simulink model "testrig_toe_camber_caster_kpi"  (R2024b)
settings: Solver=ode23t  StartTime=0.0  StopTime=309  MaxStep=0.01  RelTol=1e-3  AbsTol=1e-3  EnableMultiTasking=on
PostLoadFcn:
  | Maneuver = MDatabase.KnC.Sedan_HambaLG;
values from neighbouring files (symbols this model uses):
  Vehicle = evalin('base','Vehicle')    [sm_car_knc_plot1toecamber.m]    (also in testrig_quarter_car_results.m = sm_car_vehcfg_setPeopleOnOff(Vehicle,[0 0 0 0 0],'SuspA1'))
undefined symbols (not defined in the file or in its folder): X, Y, Z
libraries: sm_lib x12, sm_car_testrig_utilities_lib x5, nesl_utility x3, Suspension_Utilities x1
settings Model: Creator=smiller  LastModifiedBy=smiller
settings SolverCC: AutoScaleAbsTol=off  AlgebraicLoopSolver=TrustRegion  MaxZcPerStep=1
settings DataIOCC: LimitDataPoints=on  MaxDataPoints=10000  ReturnWorkspaceOutputs=off  SignalLoggingName=logsout_sm_car_testrig_quarter_car
settings OptimizationCC: LifeSpan=inf
settings DebuggingCC: UnconnectedInputMsg=warning  UnconnectedOutputMsg=warning  UnconnectedLineMsg=warning  AllowSymbolicDim=off  SFUnexpectedBacktrackingDiag=warning  SFNoUnconditionalDefaultTransitionDiag=warning  SFExecutionAtInitializationDiag=none  ArithmeticOperatorsInVariantConditions=warning
settings ModelReferenceCC: EnableRefExpFcnMdlSchedulingChecks=on
settings SFSimCC: SimUseLocalCustomCode=off  CustomCodeUndefinedFunction=UseInterfaceOnly
settings RTWCC: RTWUseLocalCustomCode=off  GPUComputeCapability=3.5  DLArmComputeVersion=19.05
settings CodeAppCC: StateflowObjectComments=on
settings GRTTargetCC: TargetLangStandard=C89/C90 (ANSI)
settings ConfigComp: CovMetricSettings=dw  CovSaveCumulativeToWorkspaceVar=on  CovSaveSingleToWorkspaceVar=on  CovExternalEMLEnable=off  CovSFcnEnable=off
settings SimscapeCC: SimscapeLogType=all  SimscapeLogSimulationStatistics=on  SimscapeLogName=simlog_sm_car_testrig_quarter_car  SimscapeLogLimitData=off  SimscapeLogDataHistory=10000
settings ExplorerConfigSet: InternalSimMechanicsExplorerSettings="<ExplorerConfiguration><canonicalview>default</canonicalview><AnimationSetting><BasePlaybackSpeed>1.0</BasePlaybackSpeed><PlaybackSpeedFactor>16.0</PlaybackSpeedFactor></AnimationSetting><TilePanel><TileInfo><Tiles Columns=\"2\" Count=\"4\" Rows=\"2\"><Column Weight=\"0.4994\"/><Column Weight=\"0.5006\"/><Row Weight=\"0.5\"/><Row Weight=\"0.5\"/><Tile Height=\"1\" Width=\"1\" X=\"0\" Y=\"0\"/><Tile Height=\"1\" Width=\"1\" X=\"0\" Y=\"1\"/><Tile Height=\"1\" Width=\"1\" X=\"1\" Y=\"0\"/><Tile Height=\"1\" Width=\"1\" X=\"1\" Y=\"1\"/></Tiles></TileInfo><SceneInfo><SceneViewer><BGColor><R>0.60000002384185791</R><G>0.60000002384185791</G><B>0.60000002384185791</B></BGColor><Camera><DoPerspective>off</DoPerspective><Position><X>0.0501116369779495557</X><Y>-0.960439324378967063</Y><Z>0.354613588377279798</Z></Position><Center><X>0.0501116369779495557</X><Y>0.0395606756210328814</Y><Z>0.354613588377279798</Z></Center><Up><X>0</X><Y>-0</Y><Z>1</Z></Up><ViewLimDist>1</ViewLimDist><YLim>0.40234222266736086</YLim><XLim>0.499223494414459068</XLim></Camera></SceneViewer><SceneViewer><BGColor><R>0.60000002384185791</R><G>0.60000002384185791</G><B>0.60000002384185791</B></BGColor><Camera><DoPerspective>off</DoPerspective><Position><X>0.0558602008410402223</X><Y>0.0302894181578547521</Y><Z>1.3621428683400163</Z></Position><Center><X>0.0558602008410402223</X><Y>0.0302894181578547521</Y><Z>0.3621428683400163</Z></Center><Up><X>0</X><Y>1</Y><Z>-0</Z></Up><ViewLimDist>1</ViewLimDist><YLim>0.294722497360931923</YLim><XLim>0.365689670946425405</XLim></Camera></SceneViewer><SceneViewer><BGColor><R>0.60000002384185791</R><G>0.60000002384185791</G><B>0.60000002384185791</B></BGColor><Camera><DoPerspective>off</DoPerspective><Position><X>1.06385555863380432</X><Y>0.0520493272308068522</Y><Z>0.359920288840733016</Z></Position><Center><X>0.0638555586338043213</X><Y>0.0520493272308068522</Y><Z>0.359920288840733016</Z></Center><Up><X>-0</X><Y>0</Y><Z>1</Z></Up><ViewLimDist>1</ViewLimDist><YLim>0.366723158690145656</YLim><XLim>0.457105353608113552</XLim></Camera></SceneViewer><SceneViewer><BGColor><R>0.60000002384185791</R><G>0.60000002384185791</G><B>0.60000002384185791</B></BGColor><Camera><DoPerspective>off</DoPerspective><Position><X>0.641205847469371593</X><Y>-0.512509662079820627</Y><Z>0.9394931381375351</Z></Position><Center><X>0.0638555782797458199</X><Y>0.0648406071098051595</Y><Z>0.362142868947909313</Z></Center><Up><X>-0.408248290463863073</X><Y>0.408248290463863073</Y><Z>0.816496580927726145</Z></Up><ViewLimDist>1</ViewLimDist><YLim>0.425868621668497427</YLim><XLim>0.530827743722772971</XLim></Camera></SceneViewer></SceneInfo></TilePanel><MechEditorPanel><Cameras/><GfxPanelCameraMap/><VideoCreator><PlaybackSpeedRatio>1.0</PlaybackSpeedRatio><FrameRate>30</FrameRate><VideoFormat>Motion JPEG AVI</VideoFormat><FrameSize>auto</FrameSize></VideoCreator></MechEditorPanel></ExplorerConfiguration>"

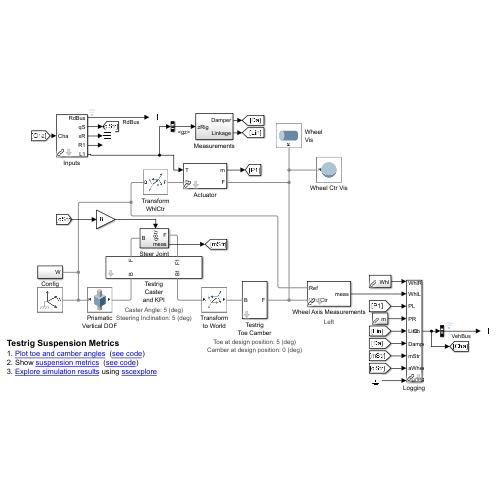
[thumbnail: Simulink's stored preview of the top-level diagram]
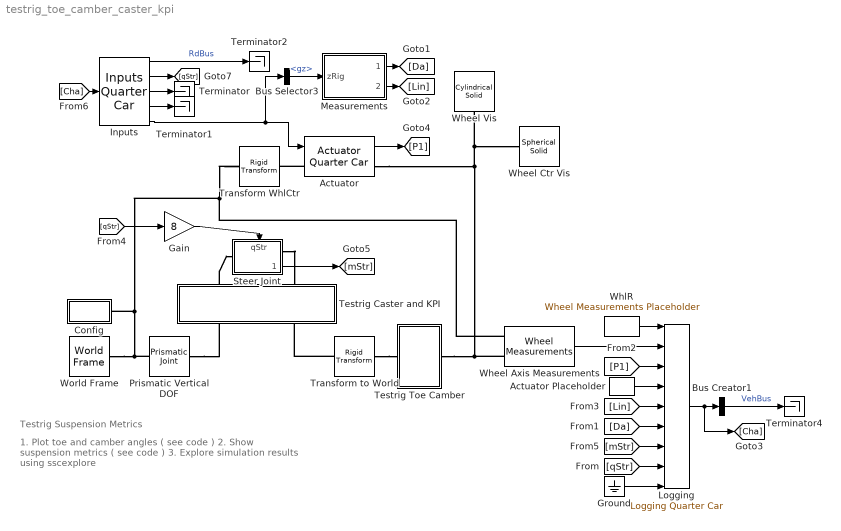
== system testrig_toe_camber_caster_kpi ==
  note: Testrig Suspension Metrics
  note: 1. Plot toe and camber angles ( see code )
      | 2. Show suspension metrics ( see code )
      | 3. Explore simulation results using sscexplore
  Actuator : sm_car_testrig_utilities_lib/Actuator Quarter Car  veh=Vehicle  xCPOffset=Maneuver.xCPOffset
  Actuator Placeholder : sm_car_testrig_utilities_lib/Actuator Placeholder  SystemSampleTime=-1  VariantActivationTime=update diagram  AllowFlexibleInterface=on  Latency=0  AutoFrameSizeCalculation=off
  Bus Creator1 : BusCreator  Inputs=1
  Bus Selector3 : BusSelector  OutputSignals=gz
  Config : Subsystem
  Gain : Gain  Gain=8
  Ground : Ground
  Inputs : sm_car_testrig_utilities_lib/Inputs Quarter Car  popup_steering_input=On
  Logging : sm_car_testrig_utilities_lib/Logging Quarter Car
  Measurements : Subsystem
  Prismatic Vertical DOF : sm_lib/Joints/Prismatic Joint  JointMode=Normal  CompositeWrenchDir=FollowerOnBase  CompositeWrenchFrame=BaseFrame  SenseConstraintForce=off  SenseConstraintTorque=off  SenseTotalForce=off  SenseTotalTorque=off  PositionTargetSpecify=off  PositionTargetPriority=High  PositionTargetValue=0  PositionTargetValueUnits=m  VelocityTargetSpecify=off  VelocityTargetPriority=High  VelocityTargetValue=0  VelocityTargetValueUnits=m/s  EquilibriumPosition=0  EquilibriumPositionUnits=m  SpringStiffness=0  SpringStiffnessUnits=N/m  DampingCoefficient=0  DampingCoefficientUnits=N/(m/s)  LowerLimitSpecify=off  LowerLimitBound=-1  LowerLimitBoundUnits=m  LowerLimitStiffness=1e6  LowerLimitStiffnessUnits=N/m  LowerLimitDamping=1e3  LowerLimitDampingUnits=N/(m/s)  LowerLimitTransitionRegionWidth=1e-4  LowerLimitTransitionRegionWidthUnits=m  UpperLimitSpecify=off  UpperLimitBound=1  UpperLimitBoundUnits=m  UpperLimitStiffness=1e6  UpperLimitStiffnessUnits=N/m  UpperLimitDamping=1e3  UpperLimitDampingUnits=N/(m/s)  UpperLimitTransitionRegionWidth=1e-4  UpperLimitTransitionRegionWidthUnits=m  TorqueActuationMode=NoTorque  MotionActuationMode=ComputedMotion  SensePosition=off  SenseVelocity=off  SenseAcceleration=off  SenseTorqueForce=off  SenseLowerLimitTorqueForce=off  SenseUpperLimitTorqueForce=off
  Steer Joint : Subsystem
      settings: PortSchema="{\"entries\":[{\"content\":{\"sides\":[{\"content\":{\"connectorIds\":[\"LConn1\"]},\"type\":\"ConnectorPlacement.EquallySpacedRectSide\",\"uuid\":\"c6bcf25b-d906-4954-990b-54daf7e75c46\"},{\"content\":{\"connectorIds\":[\"RConn1\",\"Out1\"],\"side\":\"RIGHT\"},\"type\":\"ConnectorPlacement.EquallySpacedRectSide\",\"uuid\":\"9db478a6-4a36-4e7a-9741-5384e6e9f750\"},{\"content\":{\"connectorIds\":[\"In1\"],\"side\":\"TOP\"},\"type\":\"ConnectorPlacement.EquallySpacedRectSide\",\"uuid\":\"2b79d805-6701-4165-ad8a-4e92c45830ed\"}]},\"type\":\"ConnectorPlacement.EquallySpacedConnector\",\"uuid\":\"b1957e60-a576-4b18-8f80-c65f81ef8247\"}],\"packageUris\":[\"http://schema.mathworks.com/mf0/Connector/R2020b\"],\"version\":\"1.0\"}"
  Terminator{,1..2,4} (4 alike) : Terminator
  Testrig Caster and KPI : Subsystem  mask{qCaster=5, qKP=5, xStrAxis=-0.1}
      mask prompts: qCaster "Caster Angle (deg)"; qKP "Kingpin Angle (deg)"; xStrAxis "Offset WC Steer axis"
      settings: AttributesFormatString=|
      | Caster Angle: %<qCaster> (deg)
      | Steering Inclination: %<qKP> (deg)
  Testrig Toe Camber : Subsystem  mask{qToe=5, qCamber=0}
      mask prompts: qToe "Toe"; qCamber "Camber"
      settings: AttributesFormatString=|
      | Toe at design position: %<qToe> (deg)
      | Camber at design position: %<qCamber> (deg)
  Transform WhlCtr : sm_lib/Frames and Transforms/Rigid Transform  RotationMethod=None  FollAlignAxisA=+X  BaseAlignAxisA=+Y  FollAlignAxisB=+Y  BaseAlignAxisB=+Z  RotationStandardAxis=+Z  RotationAngle=0.0  RotationAngleUnits=deg  RotationArbitraryAxis=[0 0 1]  RotationSequenceAxes=FollowerAxes  RotationSequence=XYX  RotationSequenceAngles=[0 0 0]  RotationSequenceAnglesUnits=deg  RotationMatrix=[1 0 0; 0 1 0; 0 0 1]  Quaternion=[1 0 0 0]  TranslationMethod=StandardAxis  TranslationCartesianOffset=[0 0 0]  TranslationCartesianOffsetUnits=m  TranslationStandardAxis=+Z  TranslationStandardOffset=Vehicle.Chassis.SuspA1.Linkage.Upright.sWheelCentre.Value(3)  TranslationStandardOffsetUnits=m  TranslationROffset=0  TranslationROffsetUnits=m  TranslationThetaOffset=0  TranslationThetaOffsetUnits=deg  TranslationZOffset=0  TranslationZOffsetUnits=m
  Transform to World : sm_lib/Frames and Transforms/Rigid Transform  RotationMethod=StandardAxis  FollAlignAxisA=+X  BaseAlignAxisA=+Y  FollAlignAxisB=+Y  BaseAlignAxisB=+Z  RotationStandardAxis=+X  RotationAngle=-90  RotationAngleUnits=deg  RotationArbitraryAxis=[0 0 1]  RotationSequenceAxes=FollowerAxes  RotationSequence=XYX  RotationSequenceAngles=[0 0 0]  RotationSequenceAnglesUnits=deg  RotationMatrix=[1 0 0; 0 1 0; 0 0 1]  Quaternion=[1 0 0 0]  TranslationMethod=StandardAxis  TranslationCartesianOffset=[0 0 0]  TranslationCartesianOffsetUnits=m  TranslationStandardAxis=+Z  TranslationStandardOffset=0  TranslationStandardOffsetUnits=m  TranslationROffset=0  TranslationROffsetUnits=m  TranslationThetaOffset=0  TranslationThetaOffsetUnits=deg  TranslationZOffset=0  TranslationZOffsetUnits=m
  Wheel Vis : sm_lib/Body Elements/Cylindrical Solid  CylinderRadius=Vehicle.Chassis.SuspA1.Linkage.Upright.sWheelCentre.Value(3)  CylinderRadiusUnits=m  CylinderLength=0.05  CylinderLengthUnits=m  ExportEntireGeometry=off  InertiaType=CalculateFromGeometry  BasedOnType=Density  Density=1000  DensityUnits=kg/m^3  Mass=1  MassUnits=kg  CenterOfMass=[0 0 0]  CenterOfMassUnits=m  MomentsOfInertia=[1 1 1]  MomentsOfInertiaUnits=kg*m^2  ProductsOfInertia=[0 0 0]  ProductsOfInertiaUnits=kg*m^2  GraphicType=FromGeometry  MarkerShape=Sphere  MarkerSize=10  GraphicVisPropType=SimpleVisualProperties  GraphicDiffuseColor=[0.5 0.5 0.5]  GraphicOpacity=1.0  GraphicSpecularColor=[0.5 0.5 0.5 1.0]  GraphicAmbientColor=[0.15 0.15 0.15 1.0]  GraphicEmissiveColor=[0.0 0.0 0.0 1.0]  GraphicShininess=75  DoExposeReferenceFrame=on  SerializedFrames=<Frames/>
  Wheel Axis Measurements : Suspension_Utilities/Wheel Measurements  popup_leftRight=Left
      settings: AttributesFormatString=%<popup_leftRight>
  Wheel Ctr Vis : sm_lib/Body Elements/Spherical Solid  SphereRadius=0.01  SphereRadiusUnits=m  ExportEntireGeometry=off  InertiaType=CalculateFromGeometry  BasedOnType=Density  Density=1000  DensityUnits=kg/m^3  Mass=1  MassUnits=kg  CenterOfMass=[0 0 0]  CenterOfMassUnits=m  MomentsOfInertia=[1 1 1]  MomentsOfInertiaUnits=kg*m^2  ProductsOfInertia=[0 0 0]  ProductsOfInertiaUnits=kg*m^2  GraphicType=FromGeometry  MarkerShape=Sphere  MarkerSize=10  GraphicVisPropType=SimpleVisualProperties  GraphicDiffuseColor=[0.5 0.5 0.5]  GraphicOpacity=1.0  GraphicSpecularColor=[0.5 0.5 0.5 1.0]  GraphicAmbientColor=[0.15 0.15 0.15 1.0]  GraphicEmissiveColor=[0.0 0.0 0.0 1.0]  GraphicShininess=75  DoExposeReferenceFrame=on  SerializedFrames=<Frames/>
  WhlR : sm_car_testrig_utilities_lib/Wheel Measurements Placeholder  SystemSampleTime=-1  VariantActivationTime=update diagram  AllowFlexibleInterface=on  Latency=0  AutoFrameSizeCalculation=off
  World Frame : sm_lib/Frames and Transforms/World Frame
  wires:
  Measurements/1(Damper) -> [Da]
  Measurements/2(Linkage) -> [Lin]
  Logging/1 -> [Cha], Bus Creator1/1
  Bus Creator1/1 -> Terminator4/1  "VehBus"
  Actuator/1 -> [P1]
  Gain/1 -> Steer Joint/1(qStr)
  Inputs/1 -> Terminator2/1  "RdBus"
  Inputs/3 -> Terminator/1
  Inputs/4 -> Terminator1/1
  [Cha] -> Inputs/1
  Inputs/2 -> [qStr]
  Inputs/5 -> Actuator/1, Bus Selector3/1
  Bus Selector3/1 -> Measurements/1(zRig)  "<gz>"
  [qStr] -> Gain/1
  Ground/1 -> Logging/9
  [Lin] -> Logging/5
  [mStr] -> Logging/7
  [Da] -> Logging/6
  [P1] -> Logging/3
  Wheel Axis Measurements/1 -> Logging/2
  WhlR/1 -> Logging/1
  [qStr] -> Logging/8
  Actuator Placeholder/1 -> Logging/4
  Steer Joint/1(meas) -> [mStr]
  connections:
  Wheel Vis/RConn1 -- Actuator/RConn1 -- Wheel Axis Measurements/LConn2 -- Testrig Toe Camber/RConn1 -- Wheel Ctr Vis/RConn1
  Transform to World/RConn1 -- Testrig Toe Camber/LConn1
  Steer Joint/RConn1 -- Testrig Caster and KPI/RConn2
  Testrig Caster and KPI/RConn1 -- Steer Joint/LConn1
  Transform to World/LConn1 -- Testrig Caster and KPI/LConn2
  Prismatic Vertical DOF/RConn1 -- Testrig Caster and KPI/LConn1
  Actuator/LConn1 -- Transform WhlCtr/RConn1
  World Frame/RConn1 -- Wheel Axis Measurements/LConn1 -- Transform WhlCtr/LConn1 -- Config/RConn1 -- Prismatic Vertical DOF/LConn1

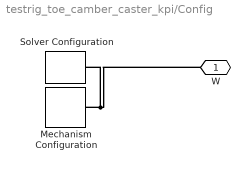
== system testrig_toe_camber_caster_kpi/Config ==
  Mechanism Configuration : sm_lib/Utilities/Mechanism Configuration  UniformGravity=Constant  GravityVector=[0 0 -9.80665]  GravityVectorUnits=m/s^2  LinearizationDelta=0.001  JointModeTransitionNonlinearIterations=2
  Solver Configuration : nesl_utility/Solver Configuration  PhysicalDomain=network_engine_domain  SubClassName=solver  LeftPortType=input  RightPortType=generic  Tones=[]  Harmonics=[]  SimulateNoise=off  Profile=off  UseLocalSampling=off  EnableSwitchedLinearOptims=on  FrequencyDomain=off  UseCCode=off  RelTol=0.001  AbsTol=1e-06  MinStep=1e-09  ToWorkspace=off  RevertToSquareIcSolve=off  NumHomotopyIterations=100  PhasorMode=off  PhasorModeNumHarmonics=1  ConsistencySolver=NEWTON_FTOL  IndexReductionMethod=DerivativeReplacement  DoDC=off  ResidualTolerance=1e-09  ConsistencyTolSource=GLOBAL  ConsistencyAbsTol=0.001  ConsistencyRelTol=0.001  ConsistencyTolFactor=0.001  UseLocalSolver=off  LocalSolverChoice=NE_BACKWARD_EULER_ADVANCER  ResolveIndetEquations=on  FunctionEvalNumThread=1  LocalSolverSampleTime=0.001  DoFixedCost=off  MaxNonlinIter=3  MaxModeIter=2  ComputeImpulses=off  ImpulseIterations=2  LinearAlgebra=Sparse  LinearAlgebraNumThread=0  EquationFormulation=NE_TIME_EF  DelaysMemoryBudget=1024  AutomaticFiltering=on  FilteringTimeConstant=0.001  PartitionStorageMethod=AS_NEEDED  PartitionMemoryBudget=1024  PartitionMethod=FAST  MultibodyUseLocalSolver=off  MultibodyLocalSolverChoice=ODE1  MultibodyLocalSolverSampleTime=0.001
  W : PMIOPort  Side=Right
  connections:
  Mechanism Configuration/RConn1 -- W/RConn1 -- Solver Configuration/RConn1

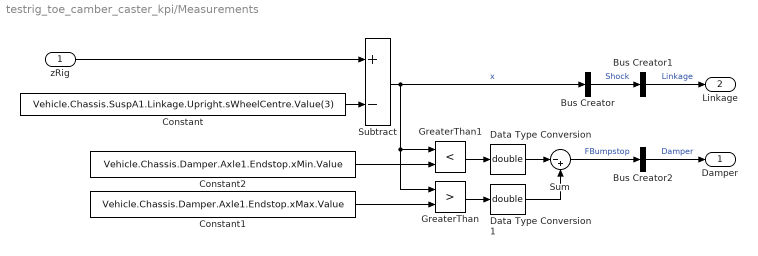
== system testrig_toe_camber_caster_kpi/Measurements ==
  zRig : Inport
  Bus Creator : BusCreator  Inputs=1
  Bus Creator1 : BusCreator  Inputs=1
  Bus Creator2 : BusCreator  Inputs=1
  Constant : Constant  Value=Vehicle.Chassis.SuspA1.Linkage.Upright.sWheelCentre.Value(3)
  Constant1 : Constant  Value=Vehicle.Chassis.Damper.Axle1.Endstop.xMax.Value
  Constant2 : Constant  Value=Vehicle.Chassis.Damper.Axle1.Endstop.xMin.Value
  Data Type Conversion : DataTypeConversion  OutDataTypeStr=double  SaturateOnIntegerOverflow=off  RndMeth=Floor
  Data Type Conversion1 : DataTypeConversion  OutDataTypeStr=double  SaturateOnIntegerOverflow=off  RndMeth=Floor
  GreaterThan : RelationalOperator  Operator=>  OutDataTypeStr=boolean  RndMeth=Simplest  InputSameDT=off
  GreaterThan1 : RelationalOperator  Operator=<  OutDataTypeStr=boolean  RndMeth=Simplest  InputSameDT=off
  Subtract : Sum  Inputs=+-
  Sum : Sum  Inputs=|-+
  Damper : Outport
  Linkage : Outport  Port=2
  wires:
  Subtract/1 -> Bus Creator/1, GreaterThan/1, GreaterThan1/1  "x"
  Bus Creator/1 -> Bus Creator1/1  "Shock"
  Data Type Conversion/1 -> Sum/1
  Data Type Conversion1/1 -> Sum/2
  Constant/1 -> Subtract/2
  GreaterThan/1 -> Data Type Conversion1/1
  Constant1/1 -> GreaterThan/2
  Constant2/1 -> GreaterThan1/2
  Sum/1 -> Bus Creator2/1  "FBumpstop"
  GreaterThan1/1 -> Data Type Conversion/1
  zRig/1 -> Subtract/1
  Bus Creator1/1 -> Linkage/1  "Linkage"
  Bus Creator2/1 -> Damper/1  "Damper"

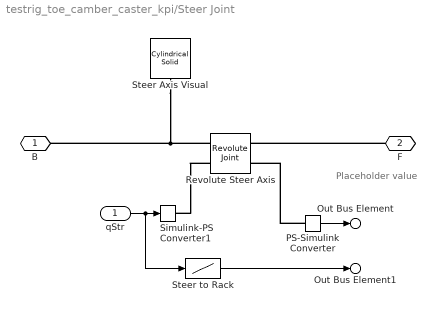
== system testrig_toe_camber_caster_kpi/Steer Joint ==
  note: Placeholder value
  qStr : Inport
  PS-Simulink Converter : nesl_utility/PS-Simulink Converter  PhysicalDomain=network_engine_domain  SubClassName=ps_output  LeftPortType=input  RightPortType=output  PseudoPeriodic=off  Frequencies=[]  VectorFormat=inherit  Unit=inherit  AffineConversion=off
  Revolute Steer Axis : sm_lib/Joints/Revolute Joint  JointMode=Normal  CompositeWrenchDir=FollowerOnBase  CompositeWrenchFrame=BaseFrame  SenseConstraintForce=off  SenseConstraintTorque=off  SenseTotalForce=off  SenseTotalTorque=off  PositionTargetSpecify=off  PositionTargetPriority=High  PositionTargetValue=0  PositionTargetValueUnits=deg  VelocityTargetSpecify=off  VelocityTargetPriority=High  VelocityTargetValue=0  VelocityTargetValueUnits=deg/s  EquilibriumPosition=0  EquilibriumPositionUnits=deg  SpringStiffness=0  SpringStiffnessUnits=N*m/deg  DampingCoefficient=0  DampingCoefficientUnits=N*m/(deg/s)  LowerLimitSpecify=off  LowerLimitBound=-90  LowerLimitBoundUnits=deg  LowerLimitStiffness=1e4  LowerLimitStiffnessUnits=N*m/deg  LowerLimitDamping=10  LowerLimitDampingUnits=N*m/(deg/s)  LowerLimitTransitionRegionWidth=0.1  LowerLimitTransitionRegionWidthUnits=deg  UpperLimitSpecify=off  UpperLimitBound=90  UpperLimitBoundUnits=deg  UpperLimitStiffness=1e4  UpperLimitStiffnessUnits=N*m/deg  UpperLimitDamping=10  UpperLimitDampingUnits=N*m/(deg/s)  UpperLimitTransitionRegionWidth=0.1  UpperLimitTransitionRegionWidthUnits=deg  TorqueActuationMode=ComputedTorque  MotionActuationMode=InputMotion  SensePosition=off  SenseVelocity=off  SenseAcceleration=off  SenseTorqueForce=on  SenseLowerLimitTorqueForce=off  SenseUpperLimitTorqueForce=off
  Simulink-PS Converter1 : nesl_utility/Simulink-PS Converter  PhysicalDomain=network_engine_domain  SubClassName=ps_input  LeftPortType=input  RightPortType=output  PseudoPeriodic=off  Frequencies=[]  NoiseDistribution=none  NoiseParameters=[]  Unit=deg  AffineConversion=off  FilteringAndDerivatives=filter  SimscapeFilterOrder=2  InputFilterTimeConstant=0.01  UdotUserProvided=0
  Steer Axis Visual : sm_lib/Body Elements/Cylindrical Solid  CylinderRadius=0.005  CylinderRadiusUnits=m  CylinderLength=Vehicle.Chassis.SuspA1.Linkage.Upright.sWheelCentre.Value(3)*2  CylinderLengthUnits=m  ExportEntireGeometry=off  InertiaType=CalculateFromGeometry  BasedOnType=Density  Density=1000  DensityUnits=kg/m^3  Mass=1  MassUnits=kg  CenterOfMass=[0 0 0]  CenterOfMassUnits=m  MomentsOfInertia=[1 1 1]  MomentsOfInertiaUnits=kg*m^2  ProductsOfInertia=[0 0 0]  ProductsOfInertiaUnits=kg*m^2  GraphicType=FromGeometry  MarkerShape=Sphere  MarkerSize=10  GraphicVisPropType=SimpleVisualProperties  GraphicDiffuseColor=[1.0 0.0 0.0]  GraphicOpacity=1.0  GraphicSpecularColor=[0.5 0.5 0.5 1.0]  GraphicAmbientColor=[0.15 0.15 0.15 1.0]  GraphicEmissiveColor=[0.0 0.0 0.0 1.0]  GraphicShininess=75  DoExposeReferenceFrame=on  SerializedFrames=<Frames/>
  Steer to Rack : Lookup_n-D  NumberOfTableDimensions=1  BreakpointsForDimension1=Vehicle.Chassis.SuspA1.Steer.Ratio_Table.aWheel.Value  Table=Vehicle.Chassis.SuspA1.Steer.Ratio_Table.xRack.Value  InternalRulePriority=Speed  RndMeth=Simplest
  B : PMIOPort  Side=Left
  F : PMIOPort  Port=2  Side=Right
  Out Bus Element : Outport  VectorParamsAs1DForOutWhenUnconnected=off  PortName=meas  Element=FRack
  Out Bus Element1 : Outport  VectorParamsAs1DForOutWhenUnconnected=off  PortName=meas  Element=xRack
  wires:
  qStr/1 -> Steer to Rack/1, Simulink-PS Converter1/1
  Steer to Rack/1 -> Out Bus Element1/1
  PS-Simulink Converter/1 -> Out Bus Element/1
  connections:
  F/RConn1 -- Revolute Steer Axis/RConn1
  Steer Axis Visual/RConn1 -- B/RConn1 -- Revolute Steer Axis/LConn1
  Revolute Steer Axis/LConn2 -- Simulink-PS Converter1/RConn1
  PS-Simulink Converter/LConn1 -- Revolute Steer Axis/RConn2

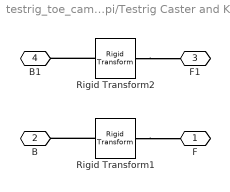
== system testrig_toe_camber_caster_kpi/Testrig Caster and KPI ==
  Rigid Transform1 : sm_lib/Frames and Transforms/Rigid Transform  RotationMethod=RotationSequence  FollAlignAxisA=+X  BaseAlignAxisA=+Y  FollAlignAxisB=+Y  BaseAlignAxisB=+Z  RotationStandardAxis=+Z  RotationAngle=0.0  RotationAngleUnits=deg  RotationArbitraryAxis=[0 0 1]  RotationSequenceAxes=FollowerAxes  RotationSequence=ZYX  RotationSequenceAngles=[0 qCaster qKP]  RotationSequenceAnglesUnits=deg  RotationMatrix=[1 0 0; 0 1 0; 0 0 1]  Quaternion=[1 0 0 0]  TranslationMethod=StandardAxis  TranslationCartesianOffset=[0 0 0]  TranslationCartesianOffsetUnits=m  TranslationStandardAxis=+Y  TranslationStandardOffset=xStrAxis  TranslationStandardOffsetUnits=m  TranslationROffset=0  TranslationROffsetUnits=m  TranslationThetaOffset=0  TranslationThetaOffsetUnits=deg  TranslationZOffset=0  TranslationZOffsetUnits=m
  Rigid Transform2 : sm_lib/Frames and Transforms/Rigid Transform  RotationMethod=RotationSequence  FollAlignAxisA=+X  BaseAlignAxisA=+Y  FollAlignAxisB=+Y  BaseAlignAxisB=+Z  RotationStandardAxis=+Z  RotationAngle=0.0  RotationAngleUnits=deg  RotationArbitraryAxis=[0 0 1]  RotationSequenceAxes=FollowerAxes  RotationSequence=ZYX  RotationSequenceAngles=[0 qCaster qKP]  RotationSequenceAnglesUnits=deg  RotationMatrix=[1 0 0; 0 1 0; 0 0 1]  Quaternion=[1 0 0 0]  TranslationMethod=StandardAxis  TranslationCartesianOffset=[0 0 0]  TranslationCartesianOffsetUnits=m  TranslationStandardAxis=+Y  TranslationStandardOffset=xStrAxis  TranslationStandardOffsetUnits=m  TranslationROffset=0  TranslationROffsetUnits=m  TranslationThetaOffset=0  TranslationThetaOffsetUnits=deg  TranslationZOffset=0  TranslationZOffsetUnits=m
  F : PMIOPort  Side=Right
  B : PMIOPort  Port=2  Side=Left
  F1 : PMIOPort  Port=3  Side=Right
  B1 : PMIOPort  Port=4  Side=Left
  connections:
  Rigid Transform1/LConn1 -- B/RConn1
  Rigid Transform1/RConn1 -- F/RConn1
  Rigid Transform2/RConn1 -- F1/RConn1
  Rigid Transform2/LConn1 -- B1/RConn1

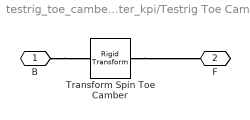
== system testrig_toe_camber_caster_kpi/Testrig Toe Camber ==
  Transform Spin Toe Camber : sm_lib/Frames and Transforms/Rigid Transform  RotationMethod=RotationSequence  FollAlignAxisA=+X  BaseAlignAxisA=+Y  FollAlignAxisB=+Y  BaseAlignAxisB=+Z  RotationStandardAxis=+Z  RotationAngle=0.0  RotationAngleUnits=deg  RotationArbitraryAxis=[0 0 1]  RotationSequenceAxes=FollowerAxes  RotationSequence=ZYX  RotationSequenceAngles=[0 qToe qCamber]  RotationSequenceAnglesUnits=deg  RotationMatrix=[1 0 0; 0 1 0; 0 0 1]  Quaternion=[1 0 0 0]  TranslationMethod=None  TranslationCartesianOffset=[0 0 0]  TranslationCartesianOffsetUnits=m  TranslationStandardAxis=+Z  TranslationStandardOffset=0  TranslationStandardOffsetUnits=m  TranslationROffset=0  TranslationROffsetUnits=m  TranslationThetaOffset=0  TranslationThetaOffsetUnits=deg  TranslationZOffset=0  TranslationZOffsetUnits=m
  B : PMIOPort  Side=Left
  F : PMIOPort  Port=2  Side=Right
  connections:
  B/RConn1 -- Transform Spin Toe Camber/LConn1
  Transform Spin Toe Camber/RConn1 -- F/RConn1
